simulink model "s_b4a4x32kf_26"  (R2018a)
settings: Solver=VariableStepDiscrete  StartTime=0.0  StopTime=10000  RelTol=1e-3
undefined symbols (not defined in the file): fft_stages, n_bits_ants, n_bits_xengs
libraries: xbsIndex_r4 x21247, casper_library_misc x37, casper_library_scopes x13, casper_library_delays x8, xbsReplacements_r4 x6, xps_library x4
(part 15 of 268)

== system s_b4a4x32kf_26/tvg_control ==
  convert1_{1..11,14..15,17..20} (17 alike) : DataTypeConversion  OutDataTypeStr=fixdt('ufix1_En0')  LockScale=on
  convert1_{12..13,16,21..23} (6 alike) : DataTypeConversion  OutDataTypeStr=fixdt('ufix2_En0')  LockScale=on
  convert2_{1..11,14..15,17..20} (17 alike) : DataTypeConversion  OutDataTypeStr=fixdt('ufix1_En0')  ConvertRealWorld=Stored Integer (SI)  LockScale=on
  convert2_{12..13,16,21..23} (6 alike) : DataTypeConversion  OutDataTypeStr=fixdt('ufix2_En0')  ConvertRealWorld=Stored Integer (SI)  LockScale=on
  gain_1 : Gain  Gain=268435456
  gain_10 : Gain  Gain=524288
  gain_11 : Gain  Gain=262144
  gain_12 : Gain  Gain=65536
  gain_13 : Gain  Gain=16384
  gain_14 : Gain  Gain=8192
  gain_15 : Gain  Gain=4096
  gain_16 : Gain  Gain=1024
  gain_17 : Gain  Gain=512
  gain_18 : Gain  Gain=256
  gain_19 : Gain  Gain=128
  gain_2 : Gain  Gain=134217728
  gain_20 : Gain  Gain=64
  gain_21 : Gain  Gain=16
  gain_22 : Gain  Gain=4
  gain_23 : Gain
  gain_3 : Gain  Gain=67108864
  gain_4 : Gain  Gain=33554432
  gain_5 : Gain  Gain=16777216
  gain_6 : Gain  Gain=8388608
  gain_7 : Gain  Gain=4194304
  gain_8 : Gain  Gain=2097152
  gain_9 : Gain  Gain=1048576
  io_delay : xbsIndex_r4/Delay  rst=off  infoeditControl=Selection of Reset will increase slice count due to use of real FFs and instead of SRLs  en=off  latency=0  reg_retiming=on  dbl_ovrd=off  block_type=delay
  reint{12..13,16,20..23} (7 alike) : xbsIndex_r4/Reinterpret  force_arith_type=on  arith_type=Unsigned  force_bin_pt=on  bin_pt=0  block_type=reinterpret
  s_b4a4x32kf_26_tvg_control_user_data_out : xbsIndex_r4/Gateway In  gui_display_data_type=Fixed-point  arith_type=Unsigned  n_bits=32  bin_pt=0  preci_type=Single  exp_width=8  frac_width=24  rows=1  columns=1  quantization="Round  (unbiased: +/- Inf)"  overflow=Saturate  period=1  UseAsADC=off  ADCChannel='1'  interface=None  automatic_assignment=on  address_offset=hex2dec('00')  intf_name=''  intf_description=''  default_value=0  timing_constraint=None  locs_specified=off  LOCs={}  io_standard={}  inherit_from_input=off  hdl_port=on  dbl_ovrd=off  block_type=gatewayin
  sim_{1..23} (23 alike) : Constant  Value=0
  sim_add : Sum  Inputs=+++++++++++++++++++++++  OutDataTypeStr=uint32
  slice_preproc_snap_dv_mux : xbsIndex_r4/Slice  nbits=1  boolean_output=on  mode=Lower Bit Location + Width  bit1=0  base1=MSB of Input  bit0=12  base0=LSB of Input  dbl_ovrd=off  block_type=slice
  slice_preproc_snap_stop_mux : xbsIndex_r4/Slice  nbits=1  boolean_output=off  mode=Lower Bit Location + Width  bit1=0  base1=MSB of Input  bit0=6  base0=LSB of Input  dbl_ovrd=off  block_type=slice
  slice_reord_snap_dv_arm : xbsIndex_r4/Slice  nbits=1  boolean_output=on  mode=Lower Bit Location + Width  bit1=0  base1=MSB of Input  bit0=13  base0=LSB of Input  dbl_ovrd=off  block_type=slice
  slice_reord_snap_dv_mux : xbsIndex_r4/Slice  nbits=2  boolean_output=off  mode=Lower Bit Location + Width  bit1=0  base1=MSB of Input  bit0=16  base0=LSB of Input  dbl_ovrd=off  block_type=slice
  slice_snap_hmc_pkt_reord_we_sel : xbsIndex_r4/Slice  nbits=2  boolean_output=off  mode=Lower Bit Location + Width  bit1=0  base1=MSB of Input  bit0=4  base0=LSB of Input  dbl_ovrd=off  block_type=slice
  slice_snap_hmc_reord_stop_sel : xbsIndex_r4/Slice  nbits=2  boolean_output=off  mode=Lower Bit Location + Width  bit1=0  base1=MSB of Input  bit0=10  base0=LSB of Input  dbl_ovrd=off  block_type=slice
  slice_snap_reord_mux_stop_sel : xbsIndex_r4/Slice  nbits=2  boolean_output=off  mode=Lower Bit Location + Width  bit1=0  base1=MSB of Input  bit0=0  base0=LSB of Input  dbl_ovrd=off  block_type=slice
  slice_snap_reord_mux_we_sel : xbsIndex_r4/Slice  nbits=2  boolean_output=off  mode=Lower Bit Location + Width  bit1=0  base1=MSB of Input  bit0=2  base0=LSB of Input  dbl_ovrd=off  block_type=slice
  slice_vacc_tvg_ctr2_en : xbsIndex_r4/Slice  nbits=1  boolean_output=on  mode=Lower Bit Location + Width  bit1=0  base1=MSB of Input  bit0=21  base0=LSB of Input  dbl_ovrd=off  block_type=slice
  slice_vacc_tvg_ctr3_en : xbsIndex_r4/Slice  nbits=1  boolean_output=on  mode=Lower Bit Location + Width  bit1=0  base1=MSB of Input  bit0=20  base0=LSB of Input  dbl_ovrd=off  block_type=slice
  slice_vacc_tvg_ctr_en : xbsIndex_r4/Slice  nbits=1  boolean_output=on  mode=Lower Bit Location + Width  bit1=0  base1=MSB of Input  bit0=22  base0=LSB of Input  dbl_ovrd=off  block_type=slice
  slice_vacc_tvg_data_sel : xbsIndex_r4/Slice  nbits=1  boolean_output=on  mode=Lower Bit Location + Width  bit1=0  base1=MSB of Input  bit0=24  base0=LSB of Input  dbl_ovrd=off  block_type=slice
  slice_vacc_tvg_pulse_en : xbsIndex_r4/Slice  nbits=1  boolean_output=on  mode=Lower Bit Location + Width  bit1=0  base1=MSB of Input  bit0=27  base0=LSB of Input  dbl_ovrd=off  block_type=slice
  slice_vacc_tvg_reset : xbsIndex_r4/Slice  nbits=1  boolean_output=on  mode=Lower Bit Location + Width  bit1=0  base1=MSB of Input  bit0=23  base0=LSB of Input  dbl_ovrd=off  block_type=slice
  slice_vacc_tvg_run : xbsIndex_r4/Slice  nbits=1  boolean_output=on  mode=Lower Bit Location + Width  bit1=0  base1=MSB of Input  bit0=18  base0=LSB of Input  dbl_ovrd=off  block_type=slice
  slice_vacc_tvg_sync_sel : xbsIndex_r4/Slice  nbits=1  boolean_output=on  mode=Lower Bit Location + Width  bit1=0  base1=MSB of Input  bit0=26  base0=LSB of Input  dbl_ovrd=off  block_type=slice
  slice_vacc_tvg_time_sel : xbsIndex_r4/Slice  nbits=1  boolean_output=on  mode=Lower Bit Location + Width  bit1=0  base1=MSB of Input  bit0=28  base0=LSB of Input  dbl_ovrd=off  block_type=slice
  slice_vacc_tvg_valid_sel : xbsIndex_r4/Slice  nbits=1  boolean_output=on  mode=Lower Bit Location + Width  bit1=0  base1=MSB of Input  bit0=25  base0=LSB of Input  dbl_ovrd=off  block_type=slice
  slice_vacc_tvg_vector_en : xbsIndex_r4/Slice  nbits=1  boolean_output=on  mode=Lower Bit Location + Width  bit1=0  base1=MSB of Input  bit0=19  base0=LSB of Input  dbl_ovrd=off  block_type=slice
  slice_xeng_tvg_data_sel : xbsIndex_r4/Slice  nbits=2  boolean_output=off  mode=Lower Bit Location + Width  bit1=0  base1=MSB of Input  bit0=14  base0=LSB of Input  dbl_ovrd=off  block_type=slice
  slice_xeng_tvg_inj_vector : xbsIndex_r4/Slice  nbits=1  boolean_output=on  mode=Lower Bit Location + Width  bit1=0  base1=MSB of Input  bit0=8  base0=LSB of Input  dbl_ovrd=off  block_type=slice
  slice_xeng_tvg_mcnt_sel : xbsIndex_r4/Slice  nbits=1  boolean_output=on  mode=Lower Bit Location + Width  bit1=0  base1=MSB of Input  bit0=7  base0=LSB of Input  dbl_ovrd=off  block_type=slice
  slice_xeng_tvg_val_sel : xbsIndex_r4/Slice  nbits=1  boolean_output=on  mode=Lower Bit Location + Width  bit1=0  base1=MSB of Input  bit0=9  base0=LSB of Input  dbl_ovrd=off  block_type=slice
  in_vacc_tvg_time_sel : Outport
  in_vacc_tvg_pulse_en : Outport  Port=2
  in_vacc_tvg_sync_sel : Outport  Port=3
  in_vacc_tvg_valid_sel : Outport  Port=4
  in_vacc_tvg_data_sel : Outport  Port=5
  in_vacc_tvg_reset : Outport  Port=6
  in_vacc_tvg_ctr_en : Outport  Port=7
  in_vacc_tvg_ctr2_en : Outport  Port=8
  in_vacc_tvg_ctr3_en : Outport  Port=9
  in_vacc_tvg_vector_en : Outport  Port=10
  in_vacc_tvg_run : Outport  Port=11
  in_reord_snap_dv_mux : Outport  Port=12
  in_xeng_tvg_data_sel : Outport  Port=13
  in_reord_snap_dv_arm : Outport  Port=14
  in_preproc_snap_dv_mux : Outport  Port=15
  in_snap_hmc_reord_stop_sel : Outport  Port=16
  in_xeng_tvg_val_sel : Outport  Port=17
  in_xeng_tvg_inj_vector : Outport  Port=18
  in_xeng_tvg_mcnt_sel : Outport  Port=19
  in_preproc_snap_stop_mux : Outport  Port=20
  in_snap_hmc_pkt_reord_we_sel : Outport  Port=21
  in_snap_reord_mux_we_sel : Outport  Port=22
  in_snap_reord_mux_stop_sel : Outport  Port=23
  wires:
  s_b4a4x32kf_26_tvg_control_user_data_out/1 -> io_delay/1
  sim_add/1 -> s_b4a4x32kf_26_tvg_control_user_data_out/1
  sim_1/1 -> convert1_1/1
  convert1_1/1 -> convert2_1/1
  convert2_1/1 -> gain_1/1
  gain_1/1 -> sim_add/1
  io_delay/1 -> slice_vacc_tvg_time_sel/1, slice_vacc_tvg_pulse_en/1, slice_vacc_tvg_sync_sel/1, slice_vacc_tvg_valid_sel/1, slice_vacc_tvg_data_sel/1, slice_vacc_tvg_reset/1, slice_vacc_tvg_ctr_en/1, slice_vacc_tvg_ctr2_en/1, slice_vacc_tvg_ctr3_en/1, slice_vacc_tvg_vector_en/1, slice_vacc_tvg_run/1, slice_reord_snap_dv_mux/1, slice_xeng_tvg_data_sel/1, slice_reord_snap_dv_arm/1, slice_preproc_snap_dv_mux/1, slice_snap_hmc_reord_stop_sel/1, slice_xeng_tvg_val_sel/1, slice_xeng_tvg_inj_vector/1, slice_xeng_tvg_mcnt_sel/1, slice_preproc_snap_stop_mux/1, slice_snap_hmc_pkt_reord_we_sel/1, slice_snap_reord_mux_we_sel/1, slice_snap_reord_mux_stop_sel/1
  slice_vacc_tvg_time_sel/1 -> in_vacc_tvg_time_sel/1
  sim_2/1 -> convert1_2/1
  convert1_2/1 -> convert2_2/1
  convert2_2/1 -> gain_2/1
  gain_2/1 -> sim_add/2
  slice_vacc_tvg_pulse_en/1 -> in_vacc_tvg_pulse_en/1
  sim_3/1 -> convert1_3/1
  convert1_3/1 -> convert2_3/1
  convert2_3/1 -> gain_3/1
  gain_3/1 -> sim_add/3
  slice_vacc_tvg_sync_sel/1 -> in_vacc_tvg_sync_sel/1
  sim_4/1 -> convert1_4/1
  convert1_4/1 -> convert2_4/1
  convert2_4/1 -> gain_4/1
  gain_4/1 -> sim_add/4
  slice_vacc_tvg_valid_sel/1 -> in_vacc_tvg_valid_sel/1
  sim_5/1 -> convert1_5/1
  convert1_5/1 -> convert2_5/1
  convert2_5/1 -> gain_5/1
  gain_5/1 -> sim_add/5
  slice_vacc_tvg_data_sel/1 -> in_vacc_tvg_data_sel/1
  sim_6/1 -> convert1_6/1
  convert1_6/1 -> convert2_6/1
  convert2_6/1 -> gain_6/1
  gain_6/1 -> sim_add/6
  slice_vacc_tvg_reset/1 -> in_vacc_tvg_reset/1
  sim_7/1 -> convert1_7/1
  convert1_7/1 -> convert2_7/1
  convert2_7/1 -> gain_7/1
  gain_7/1 -> sim_add/7
  slice_vacc_tvg_ctr_en/1 -> in_vacc_tvg_ctr_en/1
  sim_8/1 -> convert1_8/1
  convert1_8/1 -> convert2_8/1
  convert2_8/1 -> gain_8/1
  gain_8/1 -> sim_add/8
  slice_vacc_tvg_ctr2_en/1 -> in_vacc_tvg_ctr2_en/1
  sim_9/1 -> convert1_9/1
  convert1_9/1 -> convert2_9/1
  convert2_9/1 -> gain_9/1
  gain_9/1 -> sim_add/9
  slice_vacc_tvg_ctr3_en/1 -> in_vacc_tvg_ctr3_en/1
  sim_10/1 -> convert1_10/1
  convert1_10/1 -> convert2_10/1
  convert2_10/1 -> gain_10/1
  gain_10/1 -> sim_add/10
  slice_vacc_tvg_vector_en/1 -> in_vacc_tvg_vector_en/1
  sim_11/1 -> convert1_11/1
  convert1_11/1 -> convert2_11/1
  convert2_11/1 -> gain_11/1
  gain_11/1 -> sim_add/11
  slice_vacc_tvg_run/1 -> in_vacc_tvg_run/1
  sim_12/1 -> convert1_12/1
  convert1_12/1 -> convert2_12/1
  convert2_12/1 -> gain_12/1
  gain_12/1 -> sim_add/12
  slice_reord_snap_dv_mux/1 -> reint12/1
  reint12/1 -> in_reord_snap_dv_mux/1
  sim_13/1 -> convert1_13/1
  convert1_13/1 -> convert2_13/1
  convert2_13/1 -> gain_13/1
  gain_13/1 -> sim_add/13
  slice_xeng_tvg_data_sel/1 -> reint13/1
  reint13/1 -> in_xeng_tvg_data_sel/1
  sim_14/1 -> convert1_14/1
  convert1_14/1 -> convert2_14/1
  convert2_14/1 -> gain_14/1
  gain_14/1 -> sim_add/14
  slice_reord_snap_dv_arm/1 -> in_reord_snap_dv_arm/1
  sim_15/1 -> convert1_15/1
  convert1_15/1 -> convert2_15/1
  convert2_15/1 -> gain_15/1
  gain_15/1 -> sim_add/15
  slice_preproc_snap_dv_mux/1 -> in_preproc_snap_dv_mux/1
  sim_16/1 -> convert1_16/1
  convert1_16/1 -> convert2_16/1
  convert2_16/1 -> gain_16/1
  gain_16/1 -> sim_add/16
  slice_snap_hmc_reord_stop_sel/1 -> reint16/1
  reint16/1 -> in_snap_hmc_reord_stop_sel/1
  sim_17/1 -> convert1_17/1
  convert1_17/1 -> convert2_17/1
  convert2_17/1 -> gain_17/1
  gain_17/1 -> sim_add/17
  slice_xeng_tvg_val_sel/1 -> in_xeng_tvg_val_sel/1
  sim_18/1 -> convert1_18/1
  convert1_18/1 -> convert2_18/1
  convert2_18/1 -> gain_18/1
  gain_18/1 -> sim_add/18
  slice_xeng_tvg_inj_vector/1 -> in_xeng_tvg_inj_vector/1
  sim_19/1 -> convert1_19/1
  convert1_19/1 -> convert2_19/1
  convert2_19/1 -> gain_19/1
  gain_19/1 -> sim_add/19
  slice_xeng_tvg_mcnt_sel/1 -> in_xeng_tvg_mcnt_sel/1
  sim_20/1 -> convert1_20/1
  convert1_20/1 -> convert2_20/1
  convert2_20/1 -> gain_20/1
  gain_20/1 -> sim_add/20
  slice_preproc_snap_stop_mux/1 -> reint20/1
  reint20/1 -> in_preproc_snap_stop_mux/1
  sim_21/1 -> convert1_21/1
  convert1_21/1 -> convert2_21/1
  convert2_21/1 -> gain_21/1
  gain_21/1 -> sim_add/21
  slice_snap_hmc_pkt_reord_we_sel/1 -> reint21/1
  reint21/1 -> in_snap_hmc_pkt_reord_we_sel/1
  sim_22/1 -> convert1_22/1
  convert1_22/1 -> convert2_22/1
  convert2_22/1 -> gain_22/1
  gain_22/1 -> sim_add/22
  slice_snap_reord_mux_we_sel/1 -> reint22/1
  reint22/1 -> in_snap_reord_mux_we_sel/1
  sim_23/1 -> convert1_23/1
  convert1_23/1 -> convert2_23/1
  convert2_23/1 -> gain_23/1
  gain_23/1 -> sim_add/23
  slice_snap_reord_mux_stop_sel/1 -> reint23/1
  reint23/1 -> in_snap_reord_mux_stop_sel/1
